simulink model "avoidance"  (R2024b)
settings: Solver=FixedStepAuto  StartTime=0.0  StopTime=30  FixedStep=0.01  RelTol=1e-3
libraries: simulink x2, fuzblock x1
settings Model: Creator=l18  LastModifiedBy=l18

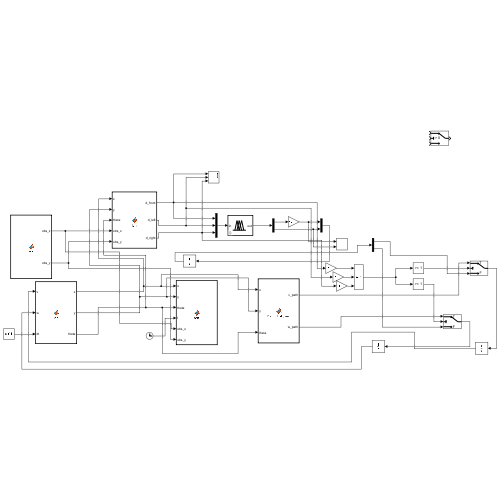
[thumbnail: Simulink's stored preview of the top-level diagram]
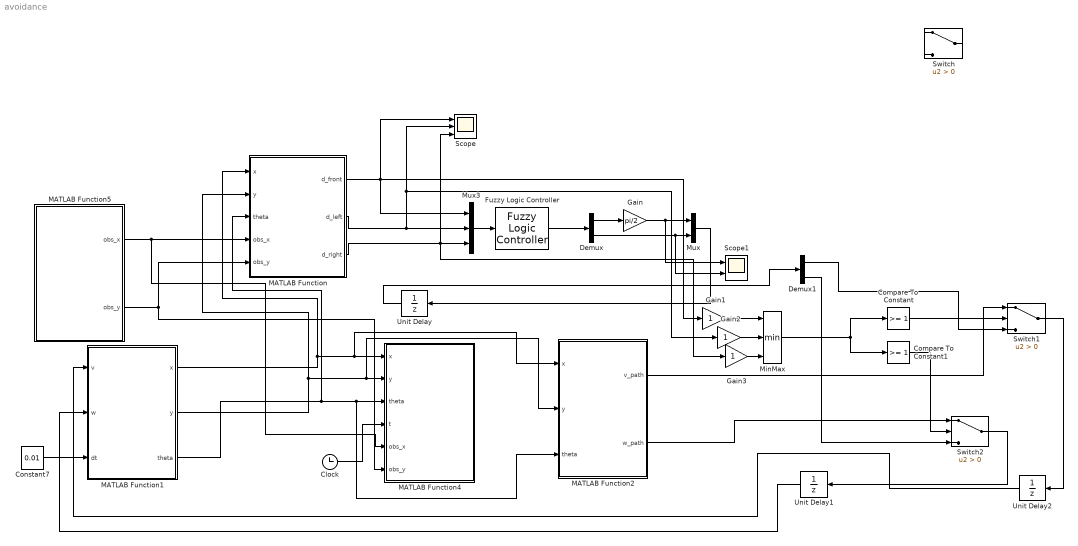
== system avoidance ==
  Clock : Clock
  Compare To Constant : simulink/Logic and Bit Operations/Compare To Constant  relop=>=  const=1  OutDataTypeStr=boolean
  Compare To Constant1 : simulink/Logic and Bit Operations/Compare To Constant  relop=>=  const=1  OutDataTypeStr=boolean
  Constant7 : Constant  Value=0.01
  Demux : Demux  Outputs=2
  Demux1 : Demux  Outputs=2
  Fuzzy Logic Controller : fuzblock/Fuzzy Logic  Controller  FIS='avoidance_v2.fis'  OutputSampleNumber=1000  DataType=double  FuzzifiedInputs=off  RuleFiringStrengths=off  RuleOutputs=off  AggregatedOutputs=off  SimulateUsing=Interpreted execution  OutOfRangeInputValueMessage=warning  NoRuleFiredMessage=warning  EmptyOutputFuzzySetMessage=warning
  Gain : Gain  Gain=pi/2
  Gain1 : Gain
  Gain2 : Gain
  Gain3 : Gain
  MATLAB Function : MATLAB Function  TreatAsAtomicUnit=on
  MATLAB Function1 : MATLAB Function  TreatAsAtomicUnit=on
  MATLAB Function2 : MATLAB Function  TreatAsAtomicUnit=on
  MATLAB Function4 : MATLAB Function  TreatAsAtomicUnit=on
  MATLAB Function5 : MATLAB Function  TreatAsAtomicUnit=on
  MinMax : MinMax  Inputs=3
  Mux : Mux  Inputs=2
  Mux3 : Mux  Inputs=3
  Scope : Scope  NumInputPorts=3
  Scope1 : Scope  NumInputPorts=2
  Switch : Switch  Criteria=u2 > Threshold  SaturateOnIntegerOverflow=off  InputSameDT=off
  Switch1 : Switch  Criteria=u2 > Threshold  SaturateOnIntegerOverflow=off  InputSameDT=off
  Switch2 : Switch  Criteria=u2 > Threshold  SaturateOnIntegerOverflow=off  InputSameDT=off
  Unit Delay : UnitDelay  SampleTime=-1  HasFrameUpgradeWarning=on
  Unit Delay1 : UnitDelay  SampleTime=-1  HasFrameUpgradeWarning=on
  Unit Delay2 : UnitDelay  SampleTime=-1  HasFrameUpgradeWarning=on
  wires:
  Fuzzy Logic Controller/1 -> Demux/1
  MATLAB Function/1(d_front) -> Gain1/1, Scope/1, Mux3/1
  MATLAB Function/2(d_left) -> Gain2/1, Scope/2, Mux3/2
  MATLAB Function/3(d_right) -> Gain3/1, Scope/3, Mux3/3
  MATLAB Function5/2(obs_y) -> MATLAB Function/5(obs_y), MATLAB Function4/6(obs_y)
  MATLAB Function1/1(x) -> MATLAB Function/1(x), MATLAB Function2/1(x), MATLAB Function4/1(x)
  MATLAB Function1/3(theta) -> MATLAB Function/3(theta), MATLAB Function2/3(theta), MATLAB Function4/3(theta)
  MATLAB Function5/1(obs_x) -> MATLAB Function4/5(obs_x), MATLAB Function/4(obs_x)
  Demux/1 -> Gain/1
  Demux/2 -> Scope1/2, Mux/2
  Mux/1 -> Unit Delay/1
  Demux1/1 -> Switch1/3
  Demux1/2 -> Switch2/3
  Constant7/1 -> MATLAB Function1/3(dt)
  Clock/1 -> MATLAB Function4/4(t)
  Unit Delay/1 -> Demux1/1
  MATLAB Function1/2(y) -> MATLAB Function/2(y), MATLAB Function2/2(y), MATLAB Function4/2(y)
  Mux3/1 -> Fuzzy Logic Controller/1
  Gain/1 -> Scope1/1, Mux/1
  MinMax/1 -> Compare To Constant1/1, Compare To Constant/1
  Compare To Constant/1 -> Switch1/2
  MATLAB Function2/1(v_path) -> Switch1/1
  Switch1/1 -> Unit Delay2/1
  MATLAB Function2/2(w_path) -> Switch2/1
  Compare To Constant1/1 -> Switch2/2
  Switch2/1 -> Unit Delay1/1
  Gain1/1 -> MinMax/1
  Gain2/1 -> MinMax/2
  Gain3/1 -> MinMax/3
  Unit Delay1/1 -> MATLAB Function1/2(w)
  Unit Delay2/1 -> MATLAB Function1/1(v)

== matlab function avoidance/MATLAB Function1 ==
  settings: sampleTime=0.01  description=小车运动模型
  data: x output; v input; y output; w input; dt input; theta output
function [x, y, theta] = fcn(v, w, dt)
    % 输入:
    %   v  : 线速度 (m/s)
    %   w  : 角速度 (rad/s)
    %   dt : 仿真步长 (s)
    
    % 使用 persistent 变量保存上一时刻的状态
    persistent x_s y_s theta_s;
    if isempty(x_s)
        x_s = 0; 
        y_s = 0;
        theta_s = 0; % 初始车头朝向设为 0
    end
    
    % --- 1. 角速度积分得到车头朝向 ---
    theta_s = theta_s + w * dt;
    
    % (可选) 将角度归一化到 [-pi, pi]，防止数值无限增大
    theta_s = atan2(sin(theta_s), cos(theta_s));
    
    % --- 2. 线速度积分得到坐标位置 ---
    x_s = x_s + v * cos(theta_s) * dt;
    y_s = y_s + v * sin(theta_s) * dt;
    
    % 输出当前时刻的状态
    x = x_s; 
    y = y_s;
    theta = theta_s;
end

== matlab function avoidance/MATLAB Function ==
  data: x input; d_front output; y input; d_left output; d_right output; theta input; obs_x input; obs_y input
function [d_front, d_left, d_right] = fcn(x, y, theta, obs_x, obs_y)
    % 设定雷达的最大探测范围（单位：米）
    % 建议改大，因为障碍物间距通常有好几米
    max_range = 1.0; 
    
    % 默认三个方向都是安全的（最大距离）
    d_front = max_range;
    d_left  = max_range;
    d_right = max_range;
   
    % ===== 核心改动：遍历所有障碍物 =====
    for i = 1:numel(obs_x)
        % 1. 计算当前障碍物的距离和角度
        dx = obs_x(i) - x;
        dy = obs_y(i) - y;
        dist = sqrt(dx^2 + dy^2);

        % 如果超出了最大探测范围，直接跳过这个障碍物
        if dist > max_range
            continue; 
        end
        
        % 计算相对角度
        rel_angle = atan2(dy, dx) - theta;
        % 归一化到 -pi 到 pi 之间
        rel_angle = atan2(sin(rel_angle), cos(rel_angle));
        
        % 2. 划分探测扇区，并更新最近距离
        % 前方：正负 45度以内 (-pi/4 到 pi/4)
        if abs(rel_angle) <= pi/4
            d_front = min(d_front, dist);
            
        % 左侧：45度 到 135度 (pi/4 到 3*pi/4)
        elseif rel_angle > pi/4 && rel_angle <= 3*pi/4
            d_left = min(d_left, dist);
            
        % 右侧：-45度 到 -135度 (-pi/4 到 -3*pi/4) —— 修正了原Bug
        elseif rel_angle < -pi/4 && rel_angle >= -3*pi/4
            d_right = min(d_right, dist);
        end
    end


    % ===== 3. 归一化处理 =====
    % 限制物理距离不超过最大探测范围，并转换到 0~1 之间
    d_front = min(d_front, max_range) / max_range;
    d_left  = min(d_left,  max_range) / max_range;
    d_right = min(d_right, max_range) / max_range;
end

== matlab function avoidance/MATLAB Function2 ==
  settings: description=生成循迹路线
  data: v_path output; w_path output; x input; y input; theta input
function [v_path, w_path] = Path_Follower(x, y, theta)
    % 预设目标点
     target_x = 10; 
     target_y = 0; 
    % 您可以在内部定义，或从外部输入
    
    % 计算目标点相对于小车的角度
    angle_to_target = atan2(target_y - y, target_x - x);
    
    % 计算角度误差
    angle_error = angle_to_target - theta;
    angle_error = atan2(sin(angle_error), cos(angle_error)); % 归一化到 [-pi, pi]
    
    % 设定预设路径的行驶速度
    v_path = 0.5; % 预设速度 (m/s)
    
    % 简单的比例控制器计算角速度
    Kp = 2.0; 
    w_path = Kp * angle_error; 
    
    % 限幅
    w_path = max(min(w_path, 1.0), -1.0);
end

== matlab function avoidance/MATLAB Function4 ==
  settings: description=小车轨迹动画显示
  data: x input; y input; theta input; t input; obs_x input; obs_y input
function fcn(x, y, theta, t, obs_x, obs_y)
    % 输入：小车状态 x, y, theta，时间 t，以及障碍物坐标 obs_x, obs_y
    persistent h_car h_trajectory h_time
    
    % 1. 初始化画布（只在仿真第一步执行）
    if isempty(h_car)
        figure('Name', 'Car Animation', 'NumberTitle', 'off');
        hold on; grid on; axis equal;
        xlabel('X (m)'); ylabel('Y (m)');
        % 根据你的轨迹和障碍物范围，建议把 xlim 和 ylim 设置大一点
        xlim([-2, 15]); ylim([-5, 5]); 
        
        % ----- 新增：画静态障碍物（红色圆形）-----
        % 如果障碍物输入是向量，这里用循环画出来
        if ~isempty(obs_x)
            theta_c = linspace(0, 2*pi, 30); % 画圆用的角度
            R = 0.3; % 假设障碍物半径为 0.3 米，你可以根据需要调整
            for i = 1:length(obs_x)
                % 填充红色圆形障碍物，边缘设为黑色
                fill(R*cos(theta_c) + obs_x(i), R*sin(theta_c) + obs_y(i), ...
                     'r', 'FaceAlpha', 0.5, 'EdgeColor', 'k');
            end
        end
        % ------------------------------------------

        % 画小车（局部坐标轮廓）
        car_x = [-0.2, 0.2, 0.2, -0.2, -0.2];
        car_y = [-0.1, -0.1, 0.1, 0.1, -0.1];
        h_car = plot(car_x + x, car_y + y, 'Color', [0.8500 0.3250 0.0980], 'LineWidth', 2); % 橙色小车更显眼
        
        % 画轨迹线
        h_trajectory = plot(x, y, 'b-', 'LineWidth', 1.5);
        
        % 创建文本对象显示时间
        h_time = text(-1.8, 4.5, 'Time: 0.00 s', 'FontSize', 12, 'FontWeight', 'bold', 'Color', 'k');
    end
    
    % 2. 计算小车当前姿态的坐标 (旋转平移)
    car_x = [-0.2, 0.2, 0.2, -0.2, -0.2];
    car_y = [-0.1, -0.1, 0.1, 0.1, -0.1];
    R = [cos(theta), -sin(theta); sin(theta), cos(theta)];
    global_coords = R * [car_x; car_y];
    new_x = global_coords(1, :) + x;
    new_y = global_coords(2, :) + y;
    
    % 3. 更新小车位置
    set(h_car, 'XData', new_x, 'YData', new_y);
    
    % 4. 更新轨迹 (把当前点追加到后面)
    set(h_trajectory, 'XData', [get(h_trajectory, 'XData'), x], ...
                      'YData', [get(h_trajectory, 'YData'), y]);
    
    % 5. 更新文本内容
    set(h_time, 'String', sprintf('Time: %.2f s', t));
    
    % 6. 强制屏幕刷新 (limitrate 能防止刷新过快导致 Simulink 卡死)
    drawnow limitrate; 
end

== matlab function avoidance/MATLAB Function5 ==
  settings: description=生成循迹路线
  data: obs_x output; obs_y output
function [obs_x, obs_y] = fcn()
    % 输出数组，即使只有一个障碍物
    obs_x = [4 1 ]; 
    obs_y = [0 1 ];
end
